simulink model "HFMA_4B_1_5_9_13"  (R2026b)
settings: Solver=FixedStepDiscrete  StopTime=stopTime  FixedStep=Ts
PreLoadFcn:
  | load('a_luts.mat')
values from neighbouring files (symbols this model uses):
  cosLUT = [1 1 1 1 1 1 1 1 1 1 1 1 ... (640 elements, 16x40)]    [iq_luts.mat]
  k_avg = 10    [Simulink_DOA_Test.m]    (also in collect_ranges.m; optimised_error_code.m)
  sinLUT = [0 0 0 0 0 0 0 0 0 0 0 0 ... (640 elements, 16x40)]    [iq_luts.mat]
  Ts = 1/8000    (= 0.000125)    [Simulink_DOA_Test.m]    (also in collect_ranges.m; optimised_error_code.m)
undefined symbols (not defined in the file or in its folder): a2_Im, a2_Re, a3_Im, a3_Re, NumBits1, NumBits2, Slope1, Slope2
libraries: hdlsllib x4, sl_signal_attributes x2
(part 6 of 6)

== system HFMA_4B_1_5_9_13/Subsystem/HFMA9/Covariance Matrix/R21/ac_bd ==
  In1 : Inport
  In2 : Inport  Port=2
  In3 : Inport  Port=3
  In4 : Inport  Port=4
  Add : Sum  OutDataTypeStr=fixdt(1,32,30)  SaturateOnIntegerOverflow=on
  Product : Product  OutDataTypeStr=fixdt(1,32,30)  SaturateOnIntegerOverflow=on
  Product1 : Product  OutDataTypeStr=fixdt(1,32,30)  SaturateOnIntegerOverflow=on
  Out1 : Outport
  wires:
  In1/1 -> Product/1
  In3/1 -> Product/2
  In2/1 -> Product1/1
  In4/1 -> Product1/2
  Product/1 -> Add/1
  Product1/1 -> Add/2
  Add/1 -> Out1/1

== system HFMA_4B_1_5_9_13/Subsystem/HFMA9/Covariance Matrix/R21/bc_ad ==
  In1 : Inport
  In2 : Inport  Port=2
  In3 : Inport  Port=3
  In4 : Inport  Port=4
  Product : Product  OutDataTypeStr=fixdt(1,32,30)  SaturateOnIntegerOverflow=on
  Product1 : Product  OutDataTypeStr=fixdt(1,32,30)  SaturateOnIntegerOverflow=on
  Subtract : Sum  Inputs=+-  OutDataTypeStr=fixdt(1,32,30)  SaturateOnIntegerOverflow=on
  Out1 : Outport
  wires:
  In2/1 -> Product/1
  In3/1 -> Product/2
  In1/1 -> Product1/1
  In4/1 -> Product1/2
  Product/1 -> Subtract/1
  Product1/1 -> Subtract/2
  Subtract/1 -> Out1/1
